simulink model "EV_powertrain_system"  (R2025b)
settings: Solver=ode23  StartTime=0.0  StopTime=Tsim  FixedStep=0.001  RelTol=1e-3
libraries: slpidlib x1
settings Model: Creator=Puki  LastModifiedBy=Puki

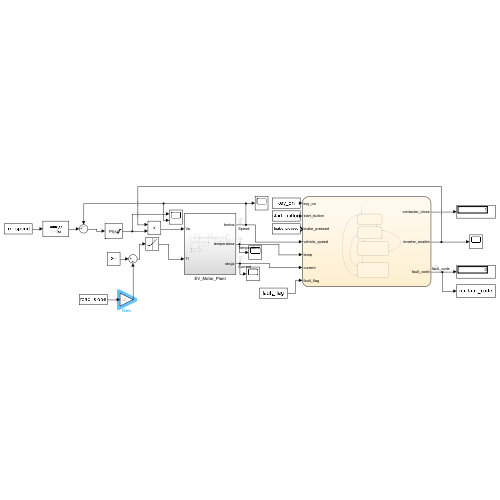
[thumbnail: Simulink's stored preview of the top-level diagram]
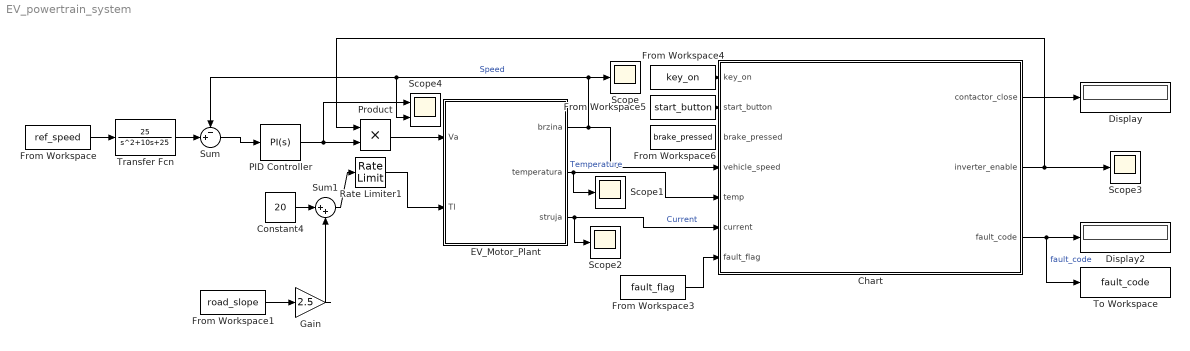
== system EV_powertrain_system ==
  Chart : Stateflow chart  TreatAsAtomicUnit=on
  Constant4 : Constant  Value=20
  Display : Display
  Display2 : Display
  EV_Motor_Plant : Subsystem
  From Workspace : FromWorkspace  VariableName=ref_speed
  From Workspace1 : FromWorkspace  VariableName=road_slope
  From Workspace3 : FromWorkspace  VariableName=fault_flag
  From Workspace4 : FromWorkspace  VariableName=key_on
  From Workspace5 : FromWorkspace  VariableName=start_button
  From Workspace6 : FromWorkspace  VariableName=brake_pressed
  Gain : Gain  Gain=2.5
  PID Controller : slpidlib/PID Controller  Controller=PI  Form=Parallel  TimeDomain=Continuous-time  UseExternalTs=off  SampleTime=-1  IntegratorMethod=Forward Euler  FilterMethod=Forward Euler  ControllerParametersSource=internal  P=0.62  I=16.6  UseKiTs=off  D=0  UseExternalDerivativeSource=off  N=100  UseFilter=on  TunerSelectOption=Transfer Function Based (PID Tuner App)  InitialConditionSource=internal  InitialConditionForIntegrator=0  InitialConditionForFilter=0  DifferentiatorICPrevScaledInput=0  ExternalReset=none  TrackingMode=off  Kt=1  LimitOutput=on  SatLimitsSource=internal  UpperSaturationLimit=160  LowerSaturationLimit=-160  LinearizeAsGain=on  AntiWindupMode=clamping  Kb=1  LimitIntegrator=off  UpperIntegratorSaturationLimit=inf  LowerIntegratorSaturationLimit=-inf  POutMin=[]  POutMax=[]  IOutMin=[]  IOutMax=[]  DOutMin=[]  DOutMax=[]  NOutMin=[]  NOutMax=[]  SumOutMin=[]  SumOutMax=[]  SaturationOutMin=[]  SaturationOutMax=[]  PParamMin=[]  PParamMax=[]  IParamMin=[]  IParamMax=[]  DParamMin=[]  DParamMax=[]  NParamMin=[]  NParamMax=[]  KbParamMin=[]  KbParamMax=[]  KtParamMin=[]  KtParamMax=[]  KbOutMin=[]  KbOutMax=[]  KtOutMin=[]  KtOutMax=[]  IntegratorOutMin=[]  IntegratorOutMax=[]  FilterOutMin=[]  FilterOutMax=[]  SumI1OutMin=[]  SumI1OutMax=[]  SumI2OutMin=[]  SumI2OutMax=[]  SumI3OutMin=[]  SumI3OutMax=[]  SumI4OutMin=[]  SumI4OutMax=[]  SumDOutMin=[]  SumDOutMax=[]  DifferentiatorOutMin=[]  DifferentiatorOutMax=[]  FilterDiffOutCoefMin=[]  FilterDiffOutCoefMax=[]  ReciprocalOutMin=[]  ReciprocalOutMax=[]  SumDenOutMin=[]  SumDenOutMax=[]  SumNumOutMin=[]  SumNumOutMax=[]  DivideOutMin=[]  DivideOutMax=[]  UdiffTsProdOutMin=[]  UdiffTsProdOutMax=[]  NTsProdOutMin=[]  NTsProdOutMax=[]  UintegralTsProdOutMin=[]  UintegralTsProdOutMax=[]  UngainTsProdOutMin=[]  UngainTsProdOutMax=[]  ClampingZeroOutDataTypeStr=Inherit: Inherit via back propagation  ClampingZeroOutMin=[]  ClampingZeroOutMax=[]  FilterDenConstantOutDataTypeStr=Inherit: Inherit via back propagation  FilterDenConstantOutMin=[]  FilterDenConstantOutMax=[]  PCopyOutDataTypeStr=Inherit: Inherit via back propagation  PCopyOutMin=[]  PCopyOutMax=[]  NCopyOutDataTypeStr=Inherit: Inherit via back propagation  NCopyOutMin=[]  NCopyOutMax=[]  IntegratorContinuousStateAttributes=''  IntegratorStateMustResolveToSignalObject=off  IntegratorRTWStateStorageClass=Auto  FilterContinuousStateAttributes=''  FilterStateMustResolveToSignalObject=off  FilterRTWStateStorageClass=Auto  ParallelPVariant=InternalParameters  IdealPVariant=Disabled  IVariant=InternalParameters  DVariant=Disabled  IntegratorVariant=Continuous  SatVariant=Enabled  AWVariant=ContClampingParallel  PCopyVariant=Disabled  TRVariant=Disabled  FdbkBlocksVariant=Forward  IdealPFdbkVariant=Disabled  SatFdbkVariant=Disabled  DerivativeFilterVariant=Disabled  NVariant=Disabled  NCopyVariant=Disabled_SignalSpec  FilterICVariant=Disabled  IntegratorICVariant=InternalICs  ExternalResetVariant=Disabled  TRSumVariant=Passthrough  SumFdbkVariant=Disabled  SumVariant=Sum_PI  TsampFilterVariant=InternalTs  TsampNgainVariant=Passthrough  TsampIntegralVariant=Disabled_SignalSpec  ExternalSaturationOutDataTypeStr=Inherit: Same as second input  DerivativeSourceVariant=Disabled  PreIntVariant=InternalPreInt
  Product : Product
  Rate Limiter1 : RateLimiter  RisingSlewLimit=15  FallingSlewLimit=-15  SampleTimeMode=inherited
  Scope{,1..3} (4 alike) : Scope
      Scope settings: ActiveDisplayYMinimum=-24.348264810782677  ActiveDisplayYMaximum=218.98794104352643  DataLoggingVariableName=Speed
      Scope1 settings: ActiveDisplayYMinimum=17.262147871084181  ActiveDisplayYMaximum=94.6406691602424  DataLoggingVariableName=Temperature
      Scope2 settings: ActiveDisplayYMinimum=-6.0216956113141666  ActiveDisplayYMaximum=54.195260501827519  DataLoggingVariableName=Current
      Scope3 settings: ActiveDisplayYMinimum=-40.760867363002731  ActiveDisplayYMaximum=4.5289852625558584  DataLoggingVariableName=ScopeData3
  Scope4 : Scope  NumInputPorts=2
      settings: ActiveDisplayYMinimum=-25.008807717293497  ActiveDisplayYMaximum=225.02912640811783  DataLoggingVariableName=ScopeData4
  Sum : Sum  Inputs=-+|
  Sum1 : Sum  Inputs=|++
  To Workspace : ToWorkspace  VariableName=fault_code  SampleTime=-1
  Transfer Fcn : TransferFcn  Numerator=[25]  Denominator=[1 10 25]
  wires:
  Chart/1(contactor_close) -> Display/1
  EV_Motor_Plant/1(brzina) -> Chart/4(vehicle_speed), Scope/1, Scope4/2, Sum/1  "Speed"
  EV_Motor_Plant/3(struja) -> Scope2/1, Chart/6(current)  "Current"
  EV_Motor_Plant/2(temperatura) -> Scope1/1, Chart/5(temp)  "Temperature"
  From Workspace3/1 -> Chart/7(fault_flag)
  Chart/3(fault_code) -> To Workspace/1, Display2/1  "fault_code"
  Chart/2(inverter_enable) -> Scope3/1, Product/1
  Sum/1 -> PID Controller/1
  PID Controller/1 -> Scope4/1, Product/2
  Product/1 -> EV_Motor_Plant/1(Va)
  Rate Limiter1/1 -> EV_Motor_Plant/2(Tl)
  From Workspace/1 -> Transfer Fcn/1
  Transfer Fcn/1 -> Sum/2
  Constant4/1 -> Sum1/1
  Sum1/1 -> Rate Limiter1/1
  Gain/1 -> Sum1/2
  From Workspace1/1 -> Gain/1
  From Workspace4/1 -> Chart/1(key_on)
  From Workspace5/1 -> Chart/2(start_button)

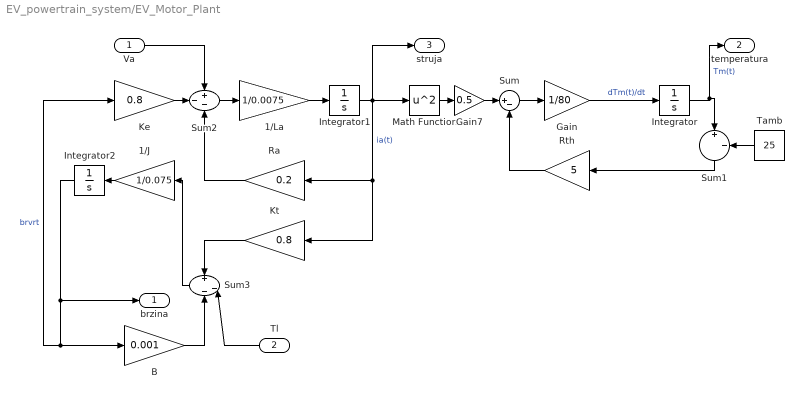
== system EV_powertrain_system/EV_Motor_Plant ==
  Va : Inport
  Tl : Inport  Port=2
  1/J : Gain  Gain=1/0.075
  1/La : Gain  Gain=1/0.0075
  B : Gain  Gain=0.001
  Gain : Gain  Gain=1/80
  Gain7 : Gain  Gain=0.5
  Integrator : Integrator  InitialCondition=25
  Integrator1 : Integrator
  Integrator2 : Integrator
  Ke : Gain  Gain=0.8
  Kt : Gain  Gain=0.8
  Math Function : Math  Operator=square
  Ra : Gain  Gain=0.2
  Rth : Gain  Gain=5
  Sum : Sum  Inputs=|+-
  Sum1 : Sum  Inputs=||+|-
  Sum2 : Sum  Inputs=+--
  Sum3 : Sum  Inputs=+|--
  Tamb : Constant  Value=25
  brzina : Outport
  temperatura : Outport  Port=2
  struja : Outport  Port=3
  wires:
  Integrator/1 -> temperatura/1, Sum1/1  "Tm(t)"
  Integrator2/1 -> brzina/1, Ke/1, B/1  "brvrt"
  1/La/1 -> Integrator1/1
  Tl/1 -> Sum3/2
  Integrator1/1 -> Math Function/1, struja/1, Kt/1, Ra/1  "ia(t)"
  B/1 -> Sum3/3
  1/J/1 -> Integrator2/1
  Ra/1 -> Sum2/3
  Sum1/1 -> Rth/1
  Rth/1 -> Sum/2
  Math Function/1 -> Gain7/1
  Tamb/1 -> Sum1/2
  Gain/1 -> Integrator/1  "dTm(t)/dt"
  Sum3/1 -> 1/J/1
  Sum/1 -> Gain/1
  Sum2/1 -> 1/La/1
  Ke/1 -> Sum2/2
  Gain7/1 -> Sum/1
  Va/1 -> Sum2/1
  Kt/1 -> Sum3/1

== stateflow chart EV_powertrain_system/Chart ==
  state Off
    entry:
    contactor_close = 0;
    inverter_enable = 0;
    fault_code = 0;
  state Standby
    entry:
    contactor_close = 1;
    inverter_enable = 0;
    fault_code = 0;
  state Drive
    entry:
    contactor_close = 1;
    inverter_enable = 1;
    fault_code = 0;
  state Fault
    entry:
    contactor_close = 0;
    inverter_enable = 0;
    fault_code = 1;
  (default) -> Off
  Off -> Fault [order 1] : [fault_flag == 1 || temp > 110 || current > 250]
  Off -> Standby [order 2] : [key_on ==1 && fault_flag == 0]
  Drive -> Standby [order 2] : [vehicle_speed == 0 && brake_pressed == 1]
  Standby -> Fault [order 1] : [fault_flag == 1 || temp > 110 || current > 250]
  Standby -> Drive [order 2] : [brake_pressed == 0 && start_button == 1]
  Drive -> Fault [order 1] : [fault_flag == 1 || temp > 110 || current > 250]
  data: key_on input; start_button input; brake_pressed input; vehicle_speed input; temp input; current input; fault_flag input; contactor_close output; inverter_enable output; fault_code output
